simulink model "WarehouseRobotSim"  (R2024b)
settings: Solver=ode4  StartTime=0.0  StopTime=inf  FixedStep=0.02  RelTol=1e-3
StopFcn:
  | try, robotVisionViewer('close'); catch, end
model workspace (MAT data in the model file):
  CameraPitchDeg = 0
  HomePose = [-20 7.3 0]
  TargetActor = "TargetBox"
  Zero = 0
  gen3 : robotics.RigidBodyTree (value not decoded)
  qStow = [0; 0; 0.261799387799; 3.14159265359; -2.26892802759; 0; 0.959931088597; 1.57079632679]
undefined symbols (not defined in the file or in its folder): Actor, setupWarehouseScene, Sim3dSensor, World
libraries: sim3dlib x8, robotmobilelib x1, simulink x1, robotsim3dlib x1, sim3dcameralib x1
settings Model: Creator=ssuga  LastModifiedBy=ssuga
settings DataIOCC: ReturnWorkspaceOutputs=off

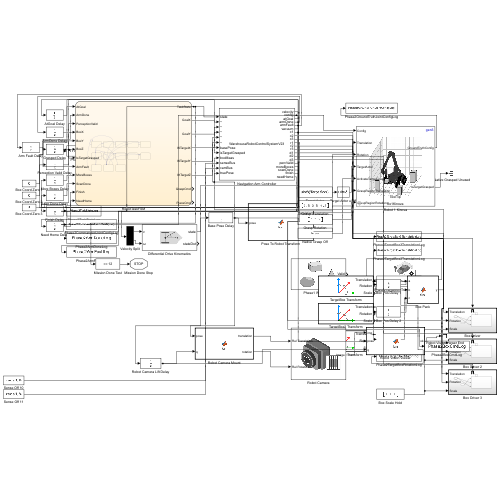
[thumbnail: Simulink's stored preview of the top-level diagram]
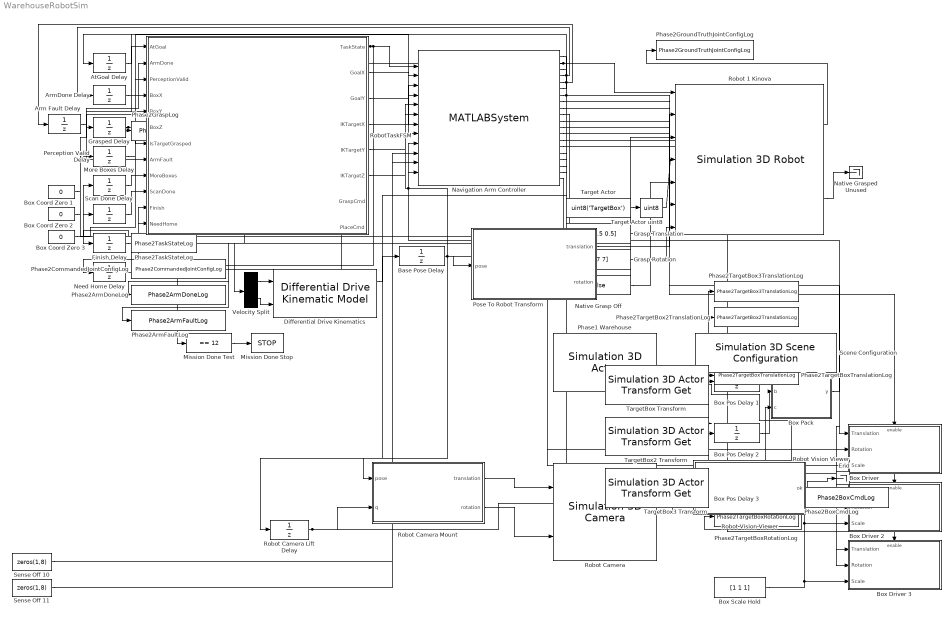
== system WarehouseRobotSim ==
  Arm Fault Delay : UnitDelay  InitialCondition=false  SampleTime=0.02  HasFrameUpgradeWarning=on
  ArmDone Delay : UnitDelay  InitialCondition=false  SampleTime=0.02  HasFrameUpgradeWarning=on
  AtGoal Delay : UnitDelay  InitialCondition=false  SampleTime=0.02  HasFrameUpgradeWarning=on
  Base Pose Delay : UnitDelay  InitialCondition=HomePose  SampleTime=0.02  HasFrameUpgradeWarning=on
  Box Coord Zero 1 : Constant  Value=0  OutDataTypeStr=double
  Box Coord Zero 2 : Constant  Value=0  OutDataTypeStr=double
  Box Coord Zero 3 : Constant  Value=0  OutDataTypeStr=double
  Box Driver : Subsystem  TreatAsAtomicUnit=on
  Box Driver 2 : Subsystem  TreatAsAtomicUnit=on
  Box Driver 3 : Subsystem  TreatAsAtomicUnit=on
  Box Pack : MATLAB Function  TreatAsAtomicUnit=on
  Box Pos Delay 1 : UnitDelay  InitialCondition=[13.225 -46.0555555555556 0.53]  SampleTime=0.02  HasFrameUpgradeWarning=on
  Box Pos Delay 2 : UnitDelay  InitialCondition=[1.725 -43.3214285714286 1.43]  SampleTime=0.02  HasFrameUpgradeWarning=on
  Box Pos Delay 3 : UnitDelay  InitialCondition=[-9.775 -43.3214285714286 2.33]  SampleTime=0.02  HasFrameUpgradeWarning=on
  Box Scale Hold : Constant  Value=[1 1 1]  VectorParams1D=off  OutDataTypeStr=double
  Differential Drive Kinematics : robotmobilelib/Differential Drive Kinematic Model  VehicleInputs=Vehicle Speed & Heading Angular Velocity  WheelRadius=0.05  WheelSpeedRange=[-inf inf]  TrackWidth=0.2  InitialState=HomePose  SimulateUsing=Interpreted execution
  Finish Delay : UnitDelay  InitialCondition=false  SampleTime=0.02  HasFrameUpgradeWarning=on
  Grasp Rotation : Constant  Value=[7 7 7]
  Grasp Translation : Constant  Value=[0.5 0.5 0.5]
  Grasped Delay : UnitDelay  InitialCondition=false  SampleTime=0.02  HasFrameUpgradeWarning=on
  Mission Done Stop : Stop
  Mission Done Test : simulink/Logic and Bit Operations/Compare To Constant  relop===  const=12  OutDataTypeStr=boolean
  More Boxes Delay : UnitDelay  InitialCondition=false  SampleTime=0.02  HasFrameUpgradeWarning=on
  Native Grasp Off : Constant  Value=false  OutDataTypeStr=boolean
  Native Grasped Unused : Terminator
  Navigation Arm Controller : MATLABSystem  System=WarehouseRobotControlSystemV23  SampleTime=0.02  RobotId=0  SimulateUsing=Interpreted execution
      mask Type: WarehouseRobotControlSystemV23
      mask Display:
      | disp('WarehouseRobotControlSystemV23');
      | port_label('input',1,'state');
      | port_label('input',2,'~');
      | port_label('input',3,'~');
      | port_label('input',4,'~');
      | port_label('input',5,'~');
      | port_label('input',6,'~');
      | port_label('input',7,'basePose');
      | port_label('input',8,'isTargetGrasped');
      | port_label('input',9,'boxMeas');
      | port_label('input',10,'senseBus');
      | port_label('input',11,'camBus');
      | port_label('input',12,'truePose');
      | port_label('output',1,'velocity');
      | port_label('output',2,'config');
      | port_label('output',3,'atGoal');
      | port_label('output',4,'armDone');
      | port_label('output',5,'armFault');
      | port_label('output',6,'vacuum');
      | port_label('output',7,'c1');
      | port_label('output',8,'c2');
      | port_label('output',9,'c3');
      | port_label('output',10,'r1');
      | port_label('output',11,'r2');
      | port_label('output',12,'r3');
      | port_label('output',13,'d1');
      | port_label('output',14,'d2');
      | port_label('output',15,'d3');
      | port_label('output',16,'percValid');
      | port_label('output',17,'moreBoxes');
      | port_label('output',18,'scanDone');
      | port_label('output',19,'finish');
      | port_label('output',20,'needHome');
  Need Home Delay : UnitDelay  InitialCondition=false  SampleTime=0.02  HasFrameUpgradeWarning=on
  Perception Valid Delay : UnitDelay  InitialCondition=false  SampleTime=0.02  HasFrameUpgradeWarning=on
  Phase1 Warehouse : sim3dlib/Simulation 3D Actor  Priority=1  ActorName=WarehouseRoot  ParentName=Scene Origin  Operation=Create at setup  InitScriptText=setupWarehouseScene(Actor,World);  SampleTime=-1  Translation=[0 0 0]  Rotation=[0 0 0]  Scale=[1 1 1]  aMode=aMode  ActorTag=WarehouseRoot  ActorType=Sim3dActor  ID=C
  Phase2ArmDoneLog : ToWorkspace  VariableName=Phase2ArmDoneLog  SaveFormat=Structure With Time  SampleTime=-1
  Phase2ArmFaultLog : ToWorkspace  VariableName=Phase2ArmFaultLog  SaveFormat=Structure With Time  SampleTime=-1
  Phase2BoxCmdLog : ToWorkspace  VariableName=Phase2BoxCmdLog  SaveFormat=Structure With Time  SampleTime=-1
  Phase2CommandedJointConfigLog : ToWorkspace  VariableName=Phase2CommandedJointConfigLog  SaveFormat=Structure With Time  SampleTime=-1
  Phase2GraspLog : ToWorkspace  VariableName=Phase2GraspLog  SaveFormat=Structure With Time  SampleTime=-1
  Phase2GroundTruthJointConfigLog : ToWorkspace  VariableName=Phase2GroundTruthJointConfigLog  SaveFormat=Structure With Time  SampleTime=-1
  Phase2TargetBox2TranslationLog : ToWorkspace  VariableName=Phase2TargetBox2TranslationLog  SaveFormat=Structure With Time  SampleTime=-1
  Phase2TargetBox3TranslationLog : ToWorkspace  VariableName=Phase2TargetBox3TranslationLog  SaveFormat=Structure With Time  SampleTime=-1
  Phase2TargetBoxRotationLog : ToWorkspace  VariableName=Phase2TargetBoxRotationLog  SaveFormat=Structure With Time  SampleTime=-1
  Phase2TargetBoxTranslationLog : ToWorkspace  VariableName=Phase2TargetBoxTranslationLog  SaveFormat=Structure With Time  SampleTime=-1
  Phase2TaskStateLog : ToWorkspace  VariableName=Phase2TaskStateLog  SaveFormat=Structure With Time  SampleTime=-1
  Pose To Robot Transform : MATLAB Function  TreatAsAtomicUnit=on
  Robot 1 Kinova : robotsim3dlib/Simulation 3D Robot  Priority=2  actorInputType=RigidBodyTree Object  RigidBodyTree=gen3  ActorName=Ro1Kinova  existActorChekBox=off  initialTrans=[0 0 0]  initialRot=[0 0 0]  initialConfig=qStow  EndEffector=ToolTip  eeOffsetInpChekBox=off  eeTargetTrans=[-0.04 0 0.245]  eeTargetRot=[0 1.2217 3.1416]  enableRegionGraspChekBox=on  regionGraspInpChekBox=on  eeTargTransDiff=[0.2 0.2 0.2]  eeTargRotDiff=[0 0 0]  inpConfEnbVal=on  inpGraspEnbVal=on  inpTransEnbVal=on  outConfEnbVal=on  outGraspEnbVal=on  outTransEnbVal=off  SampleTime=0.02  ActorType=SimulinkVehicle  ID=C  aMode=6  ActorTag=Ro1Kinova  Mesh=RigidBodyTree
  Robot Camera : sim3dcameralib/Simulation 3D Camera  Priority=1  sensorTag=Sim3dSensor�  sensorId=1  sensorName=Sim3dSensor�  vehTagList={'<empty>';'Ro1Kinova';'Scene Origin';'WarehouseRoot'}  vehTag=Scene Origin  mountLoc=Origin  offsetFlag=on  tmountOffset=[0, 0, 0]  extTmount=on  rmountOffset=[0, 0, 0]  extRmount=on  FocalLength=[300 300]  OpticalCenter=[320 240]  ImageSize=[480 640]  RadialDistortion=[0, 0]  TangentialDistortion=[0, 0]  SensorSkew=0  DepthOutportEnabled=off  SemanticOutportEnabled=off  TransformOutportEnabled=off  SampleTime=0.1  mountPoint=[0 0 0]  mountOrientation=[0 0 0]  aMode=aMode  ID=1
  Robot Camera Lift Delay : UnitDelay  InitialCondition=zeros(8,1)  SampleTime=0.02  HasFrameUpgradeWarning=on
  Robot Camera Mount : MATLAB Function  TreatAsAtomicUnit=on
  Robot Vision Viewer : MATLAB Function  TreatAsAtomicUnit=on
  Robot Vision Viewer End : Terminator
  RobotTaskFSM : Stateflow chart  TreatAsAtomicUnit=on
  Scan Done Delay : UnitDelay  InitialCondition=false  SampleTime=0.02  HasFrameUpgradeWarning=on
  Scene Configuration : sim3dlib/Simulation 3D Scene Configuration  Priority=0  ProjectFormat=Default Scenes  SceneDesc=Empty scene  ProjectName=C:\Program Files\MATLAB\R2024b\toolbox\shared\sim3d_projects\automotive_project_windows\UE\WindowsNoEditor\VehicleSimulation.exe  ScenePath=/Game/Maps/HwStrght  EnableOpenDRIVE=off  vehTagList={'Scene Origin'}  vehTag=Scene Origin  FreeCameraInitialTranslation=[0, 0, 0]  FreeCameraDefaultInitialTranslation=[-6, 0, 2]  FreeCameraInitialRotation=[0, 0, 0]  FreeCameraDefaultInitialRotation=[0, -15, 0]  OpVisEn=off  Ts=0.02  EnableWindow=on  EnableRemoteAccess=off  EnableWeather=off  SunAzimuth=90  SunAltitude=40.0  EnableGeospatialSun=off  Latitude=0  Longitude=0  Date=2023-01-01  Time=10:30:00  GeoTimeZone=-5.0  SunDaylightSaving=off  wind=1  clouds=10  EnableVolumetricClouds=off  CloudCoverage=0  CloudAltitude=6  fog=0  rain=0  RaindropsEffect=off  SnowDensity=0  EnableGeospatial=off  UseTrueOrigin=off  OriginHeight=200  OriginLatitude=40.744652  OriginLongitude=-73.988864  MapStyle=Aerial  AdditionalAssetIDs=[]  UseAdvancedSunSky=off  SolarTime=11  TimeZone=-5  Day=21  Month=9  Year=2022  UseDaylightSavingTime=on  DSTStartDay=10  DSTStartMonth=3  DSTEndDay=3  DSTEndMonth=11  DSTSwitchHour=2  sensorTag=MainCamera1  sensorId=1  sensorName=MainCamera1  mountLoc=Origin  offsetFlag=off  tmountOffset=[0, 0, 0]  rmountOffset=[0, 0, 0]  HorizontalResolution=1280  VerticalResolution=720  HorizontalFOV=60  mountPoint=[0 0 0]  mountOrientation=[0 0 0]  aMode=aMode  ID=1  GeoTrigger=Inactive
  Sense Off 10 : Constant  Value=zeros(1,8)  VectorParams1D=off  OutDataTypeStr=double
  Sense Off 11 : Constant  Value=zeros(1,8)  VectorParams1D=off  OutDataTypeStr=double
  Target Actor : Constant  Value=uint8('TargetBox')  OutDataTypeStr=uint8
  Target Actor uint8 : DataTypeConversion  OutDataTypeStr=uint8  SaturateOnIntegerOverflow=off  RndMeth=Floor
  TargetBox Transform : sim3dlib/Simulation 3D Actor Transform Get  Priority=1  ActorTag=TargetBox  NumberOfParts=1  CustNumOfParts=3  Ts=-1  aMode=aMode
  TargetBox2 Transform : sim3dlib/Simulation 3D Actor Transform Get  Priority=1  ActorTag=TargetBox2  NumberOfParts=1  CustNumOfParts=3  Ts=-1  aMode=aMode
  TargetBox3 Transform : sim3dlib/Simulation 3D Actor Transform Get  Priority=1  ActorTag=TargetBox3  NumberOfParts=1  CustNumOfParts=3  Ts=-1  aMode=aMode
  Velocity Split : Demux  Outputs=2
  wires:
  Navigation Arm Controller/3 -> AtGoal Delay/1
  AtGoal Delay/1 -> RobotTaskFSM/1(AtGoal)
  Navigation Arm Controller/4 -> ArmDone Delay/1, Phase2ArmDoneLog/1
  ArmDone Delay/1 -> RobotTaskFSM/2(ArmDone)
  Navigation Arm Controller/5 -> Arm Fault Delay/1, Phase2ArmFaultLog/1
  Arm Fault Delay/1 -> RobotTaskFSM/8(ArmFault)
  Navigation Arm Controller/16 -> Perception Valid Delay/1
  Perception Valid Delay/1 -> RobotTaskFSM/3(PerceptionValid)
  Navigation Arm Controller/17 -> More Boxes Delay/1
  More Boxes Delay/1 -> RobotTaskFSM/9(MoreBoxes)
  Navigation Arm Controller/18 -> Scan Done Delay/1
  Scan Done Delay/1 -> RobotTaskFSM/10(ScanDone)
  Navigation Arm Controller/19 -> Finish Delay/1
  Finish Delay/1 -> RobotTaskFSM/11(Finish)
  Navigation Arm Controller/20 -> Need Home Delay/1
  Need Home Delay/1 -> RobotTaskFSM/12(NeedHome)
  Box Coord Zero 1/1 -> RobotTaskFSM/4(BoxX)
  Box Coord Zero 2/1 -> RobotTaskFSM/5(BoxY)
  Box Coord Zero 3/1 -> RobotTaskFSM/6(BoxZ)
  Navigation Arm Controller/6 -> Grasped Delay/1
  Grasped Delay/1 -> RobotTaskFSM/7(IsTargetGrasped), Navigation Arm Controller/8, Phase2GraspLog/1
  TargetBox Transform/1 -> Box Pos Delay 1/1, Phase2TargetBoxTranslationLog/1
  Box Pos Delay 1/1 -> Box Pack/1(a)
  Navigation Arm Controller/7 -> Box Driver/1(Translation), Phase2BoxCmdLog/1
  Navigation Arm Controller/10 -> Box Driver/2(Rotation)
  Box Scale Hold/1 -> Box Driver/3(Scale), Box Driver 2/3(Scale), Box Driver 3/3(Scale)
  Navigation Arm Controller/13 -> Box Driver/Enable
  TargetBox2 Transform/1 -> Box Pos Delay 2/1, Phase2TargetBox2TranslationLog/1
  Box Pos Delay 2/1 -> Box Pack/2(b)
  Navigation Arm Controller/8 -> Box Driver 2/1(Translation)
  Navigation Arm Controller/11 -> Box Driver 2/2(Rotation)
  Navigation Arm Controller/14 -> Box Driver 2/Enable
  TargetBox3 Transform/1 -> Box Pos Delay 3/1, Phase2TargetBox3TranslationLog/1
  Box Pos Delay 3/1 -> Box Pack/3(c)
  Navigation Arm Controller/9 -> Box Driver 3/1(Translation)
  Navigation Arm Controller/12 -> Box Driver 3/2(Rotation)
  Navigation Arm Controller/15 -> Box Driver 3/Enable
  Box Pack/1(y) -> Navigation Arm Controller/9
  Robot 1 Kinova/2 -> Native Grasped Unused/1
  RobotTaskFSM/1(TaskState) -> Mission Done Test/1, Navigation Arm Controller/1, Phase2TaskStateLog/1
  Mission Done Test/1 -> Mission Done Stop/1
  TargetBox Transform/2 -> Phase2TargetBoxRotationLog/1
  Navigation Arm Controller/2 -> Phase2CommandedJointConfigLog/1, Robot 1 Kinova/1, Robot Camera Lift Delay/1
  Robot 1 Kinova/1 -> Phase2GroundTruthJointConfigLog/1
  RobotTaskFSM/2(GoalX) -> Navigation Arm Controller/2
  RobotTaskFSM/3(GoalY) -> Navigation Arm Controller/3
  RobotTaskFSM/4(IKTargetX) -> Navigation Arm Controller/4
  RobotTaskFSM/5(IKTargetY) -> Navigation Arm Controller/5
  RobotTaskFSM/6(IKTargetZ) -> Navigation Arm Controller/6
  Base Pose Delay/1 -> Navigation Arm Controller/7, Navigation Arm Controller/12, Pose To Robot Transform/1(pose), Robot Camera Mount/1(pose), Robot Vision Viewer/2(pose)
  Sense Off 10/1 -> Navigation Arm Controller/10
  Sense Off 11/1 -> Navigation Arm Controller/11
  Navigation Arm Controller/1 -> Velocity Split/1
  Velocity Split/1 -> Differential Drive Kinematics/1
  Velocity Split/2 -> Differential Drive Kinematics/2
  Differential Drive Kinematics/1 -> Base Pose Delay/1
  Target Actor/1 -> Target Actor uint8/1
  Pose To Robot Transform/1(translation) -> Robot 1 Kinova/2
  Pose To Robot Transform/2(rotation) -> Robot 1 Kinova/3
  Target Actor uint8/1 -> Robot 1 Kinova/4
  Native Grasp Off/1 -> Robot 1 Kinova/5
  Grasp Translation/1 -> Robot 1 Kinova/6
  Grasp Rotation/1 -> Robot 1 Kinova/7
  Robot Camera Lift Delay/1 -> Robot Camera Mount/2(q), Robot Vision Viewer/3(q)
  Robot Camera Mount/1(translation) -> Robot Camera/1
  Robot Camera Mount/2(rotation) -> Robot Camera/2
  Robot Camera/1 -> Robot Vision Viewer/1(img)
  Robot Vision Viewer/1(ok) -> Robot Vision Viewer End/1

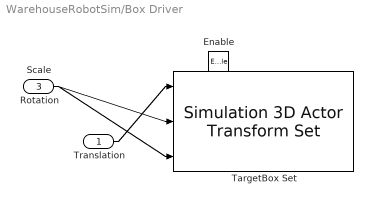
== system WarehouseRobotSim/Box Driver ==
  Translation : Inport
  Rotation : Inport  Port=2
  Scale : Inport  Port=3
  Enable : EnablePort
  TargetBox Set : sim3dlib/Simulation 3D Actor Transform Set  Priority=1  ActorTag=TargetBox  NumberOfParts=1  CustNumOfParts=3  Translation=[0 0 0]  Rotation=[0 0 0]  Scale=[1 1 1]  Ts=-1  aMode=aMode
  wires:
  Translation/1 -> TargetBox Set/1
  Rotation/1 -> TargetBox Set/2
  Scale/1 -> TargetBox Set/3

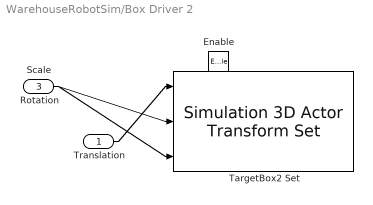
== system WarehouseRobotSim/Box Driver 2 ==
  Translation : Inport
  Rotation : Inport  Port=2
  Scale : Inport  Port=3
  Enable : EnablePort
  TargetBox2 Set : sim3dlib/Simulation 3D Actor Transform Set  Priority=1  ActorTag=TargetBox2  NumberOfParts=1  CustNumOfParts=3  Translation=[0 0 0]  Rotation=[0 0 0]  Scale=[1 1 1]  Ts=-1  aMode=aMode
  wires:
  Translation/1 -> TargetBox2 Set/1
  Rotation/1 -> TargetBox2 Set/2
  Scale/1 -> TargetBox2 Set/3

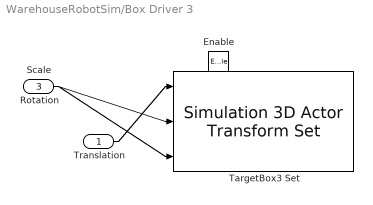
== system WarehouseRobotSim/Box Driver 3 ==
  Translation : Inport
  Rotation : Inport  Port=2
  Scale : Inport  Port=3
  Enable : EnablePort
  TargetBox3 Set : sim3dlib/Simulation 3D Actor Transform Set  Priority=1  ActorTag=TargetBox3  NumberOfParts=1  CustNumOfParts=3  Translation=[0 0 0]  Rotation=[0 0 0]  Scale=[1 1 1]  Ts=-1  aMode=aMode
  wires:
  Translation/1 -> TargetBox3 Set/1
  Rotation/1 -> TargetBox3 Set/2
  Scale/1 -> TargetBox3 Set/3

== matlab function WarehouseRobotSim/Pose To Robot Transform ==
  data: pose input; translation output; rotation output
function [translation,rotation] = fcn(pose)
% Simulation 3D expects 1-by-3 world-frame row vectors.
translation = [pose(1), pose(2), 0];
% Robot uses [yaw pitch roll]; yaw must be the first component.
rotation = [pose(3), 0, 0];

== matlab function WarehouseRobotSim/Robot Vision Viewer ==
  data: img input; ok output; pose input; q input
function ok = fcn(img,pose,q)
coder.extrinsic('robotVisionViewer');
robotVisionViewer(img,pose,q,false);
ok=uint8(0);

== matlab function WarehouseRobotSim/Box Pack ==
  data: a input; y output; b input; c input
function y = fcn(a,b,c)
% Three 1x3 carton positions (Unreal frame) -> one 1x9 controller input.
y = [a b c];

== matlab function WarehouseRobotSim/Robot Camera Mount ==
  data: pose input; translation output; q input; rotation output
function [translation,rotation] = fcn(pose,q)
% Right-handed world, yaw counter-clockwise: same heading the Robot block uses (pose(3)).
yaw=pose(3); c=cos(yaw); s=sin(yaw);
f=0.2; l=0; z=1.37+q(1);
translation=[pose(1)+f*c-l*s pose(2)+f*s+l*c z];
rotation=[0 22 1*yaw*180/pi];

== stateflow chart WarehouseRobotSim/RobotTaskFSM ==
  settings: updateMethod=DISCRETE  sampleTime=0.02
  state IDLE
    en: TaskState=uint8(0); GoalX=-20.0000; GoalY=7.3000; GraspCmd=false; PlaceCmd=false;
  state NAV_TO_STAGING
    en: TaskState=uint8(1); GoalX=15.5000; GoalY=46.0556; GraspCmd=false; PlaceCmd=false;
  state DOCK_SHELF
    en: TaskState=uint8(10); GoalX=14.1900; GoalY=46.0556; IKTargetX=BoxX; IKTargetY=BoxY; IKTargetZ=BoxZ; GraspCmd=false; PlaceCmd=false;
  state ARM_EXTEND
    en: TaskState=uint8(2); IKTargetX=BoxX; IKTargetY=BoxY; IKTargetZ=BoxZ; GraspCmd=false;
  state GRASP
    en: TaskState=uint8(3); GraspCmd=true; PlaceCmd=false;
  state ARM_RETRACT
    en: TaskState=uint8(4); GraspCmd=true; PlaceCmd=false;
  state NAV_TO_TABLE
    en: TaskState=uint8(5); GoalX=18.5000; GoalY=65.1000; GraspCmd=true;
  state ARM_PLACE
    en: TaskState=uint8(6); IKTargetX=18.5000; IKTargetY=65.9700; IKTargetZ=1.0700; GraspCmd=true;
  state RELEASE
    en: TaskState=uint8(8); GraspCmd=false; PlaceCmd=true;
  state ARM_STOW
    en: TaskState=uint8(9); GraspCmd=false; PlaceCmd=false;
  state RETURN_HOME
    en: TaskState=uint8(7); GoalX=-20.0000; GoalY=7.3000; GraspCmd=false;
  state FAULT_HOLD
    en: TaskState=uint8(11); GraspCmd=false; PlaceCmd=false;
  state MISSION_DONE
    en: TaskState=uint8(12); GoalX=-20.0000; GoalY=7.3000; GraspCmd=false; PlaceCmd=false;
  NAV_TO_STAGING -> IDLE [order 2] : [AtGoal && ScanDone && ~PerceptionValid]
  RETURN_HOME -> IDLE : [AtGoal || MoreBoxes]
  (default) -> IDLE
  GRASP -> ARM_RETRACT [order 2] : [ArmDone && IsTargetGrasped]
  DOCK_SHELF -> FAULT_HOLD [order 2] : [ArmFault]
  ARM_EXTEND -> FAULT_HOLD [order 1] : [ArmFault]
  GRASP -> FAULT_HOLD [order 1] : [ArmFault]
  IDLE -> NAV_TO_STAGING [order 1] : after(1,sec)[MoreBoxes]
  NAV_TO_STAGING -> DOCK_SHELF [order 1] : [AtGoal && ScanDone && PerceptionValid]
  DOCK_SHELF -> ARM_EXTEND [order 1] : [AtGoal && ArmDone]
  ARM_EXTEND -> GRASP [order 2] : [ArmDone]
  IDLE -> MISSION_DONE [order 3] : after(2,sec)[~MoreBoxes && Finish && ~NeedHome]
  IDLE -> RETURN_HOME [order 2] : after(1,sec)[~MoreBoxes && NeedHome]
  FAULT_HOLD -> ARM_RETRACT [order 1] : [~ArmFault && IsTargetGrasped]
  ARM_RETRACT -> NAV_TO_TABLE [order 2] : [ArmDone]
  ARM_STOW -> RETURN_HOME : [ArmDone]
  NAV_TO_TABLE -> ARM_PLACE : [AtGoal]
  ARM_PLACE -> FAULT_HOLD [order 1] : [ArmFault]
  ARM_PLACE -> RELEASE [order 2] : [ArmDone]
  FAULT_HOLD -> ARM_STOW [order 2] : [~ArmFault && ~IsTargetGrasped]
  RELEASE -> ARM_STOW [order 1] : [~IsTargetGrasped]
  RELEASE -> ARM_STOW [order 2] : after(1,sec)
  ARM_RETRACT -> FAULT_HOLD [order 1] : [ArmFault]
  data: AtGoal input boolean; ArmDone input boolean; PerceptionValid input boolean; BoxX input double; BoxY input double; BoxZ input double; IsTargetGrasped input boolean; ArmFault input boolean; MoreBoxes input boolean; ScanDone input boolean; Finish input boolean; NeedHome input boolean; TaskState output uint8; GoalX output double; GoalY output double; IKTargetX output double; IKTargetY output double; IKTargetZ output double; GraspCmd output boolean; PlaceCmd output boolean
